simulink model "ESC"  (R2026b)
settings: Solver=FixedStepAuto  StopTime=1  FixedStep=1e-6
libraries: fl_lib x21, nesl_utility x18, ee_lib x8, simulink x2, slpidlib x1, eeGeneralControl x1
settings Model: Creator=aniru  LastModifiedBy=aniru
settings DebuggingCC: AlgebraicLoopMsg=none
settings SimscapeCC: SimscapeLogType=all  SimscapeNominalValues="[{\"value\":\"1\",\"unit\":\"A\"},{\"value\":\"1\",\"unit\":\"bar\"},{\"value\":\"1\",\"unit\":\"cm^2\"},{\"value\":\"1\",\"unit\":\"cm^3/s\"},{\"value\":\"1\",\"unit\":\"kJ/kg\"},{\"value\":\"1\",\"unit\":\"kW\"},{\"value\":\"1\",\"unit\":\"l\"},{\"value\":\"1\",\"unit\":\"N\"},{\"value\":\"1\",\"unit\":\"N*m\"},{\"value\":\"1\",\"unit\":\"V\"},{\"value\":\"0.001\",\"unit\":\"Wb\"}]"  SimscapeUseEnergyAccounting=off

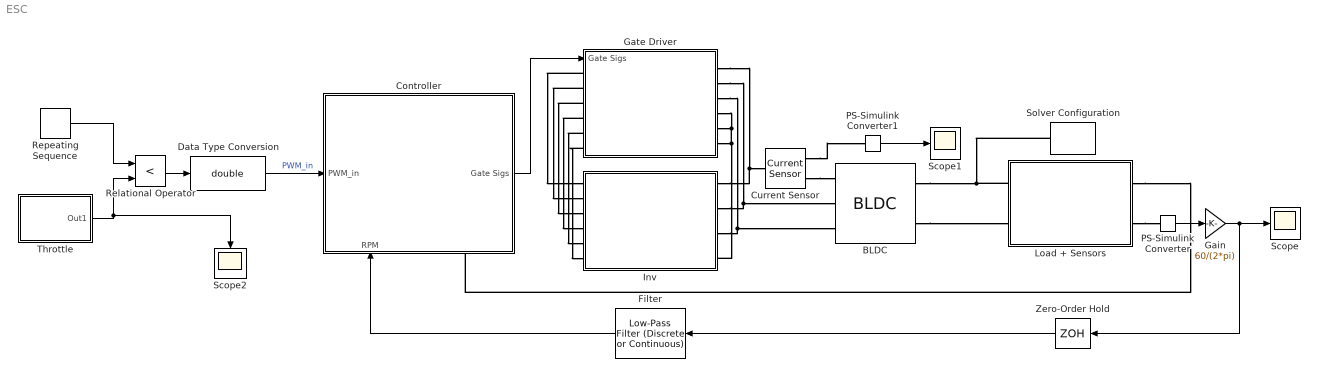
== system ESC ==
  BLDC : ee_lib/Electromechanical/Permanent Magnet/BLDC  PartSpecification="{\"CollectionId\":\"MW.SimscapeElectrical\",\"CollectionVersion\":\"1.0.0\",\"DatasetId\":\"Crouzet|80120301|simscape.electrical.bldc\",\"DisplayName\":\"Crouzet:80120301\"}"  rotor_param=ee.enum.pmsm.backemf.trapezoidflux  pm_flux_linkage=2.1333e-02 % Datasheet derived Wb  theta_constant=28.1250 % Assumed angle deg  emf_max=9.6 % Parameter not set V  w_meas=600 % Parameter not set rpm  DphiDtheta_tab=[0, -.1528, -.1528, .1528, .1528, 0] % Parameter not set Wb/rad  back_emf_tab=[0, -9.6, -9.6, 9.6, 9.6, 0] % Parameter not set V  rotor_angle_tab=[0, 7.5, 22.5, 37.5, 52.5, 60] % Parameter not set deg  nPolePairs=4 % Datasheet derived  axes_param=ee.enum.rotorangle.qaxis  port_option=ee.enum.threePhasePort.expanded  winding_type=ee.enum.electromech.statorconfiguration.wye  stator_param=ee.enum.statorparam.LdLqL0  machine_param=ee.enum.dqparameterization.constant  Ld=0.2300 % Datasheet derived mH  Lq=0.2300 % Datasheet derived mH  idVec=[-200, 0, 200] % Parameter not set A  iqVec=[-200, 0, 200] % Parameter not set A  LdMatrix=0.00022 * ones(3, 3) % Parameter not set H  LqMatrix=0.00022 * ones(3, 3) % Parameter not set H  L0=0.2300 % Assumed inductance value mH  Ls=0.0002 % Parameter not set H  Lm=0 % Parameter not set H  Ms=0.00002 % Parameter not set H  Rs=0.1000 % Datasheet derived Ohm  zero_sequence=ee.enum.park.zerosequence.exclude  loss_param=ee.enum.ironloss.none  losses_oc=[0, 0, 0] % Parameter not set W  losses_sc=[0, 0, 0] % Parameter not set W  f_losses=60 % Parameter not set Hz  Isc_losses=95 % Parameter not set A  J=1.6000e-04 % Datasheet derived kg*m^2  lam=0 % Parameter not set N*m*s/rad  i_d_specify=off  i_d_priority=None  i_d=0 A  i_d_nominal_specify=off  i_d_nominal_value=1  i_d_nominal_unit=A  i_q_specify=off  i_q_priority=None  i_q=0 A  i_q_nominal_specify=off  i_q_nominal_value=1  i_q_nominal_unit=A  torque_specify=off  torque_priority=None  torque=0 N*m  torque_nominal_specify=off  torque_nominal_value=1  torque_nominal_unit=N*m  angular_velocity_specify=off  angular_velocity_priority=High  angular_velocity=0 rpm  angular_velocity_nominal_specify=off  angular_velocity_nominal_value=1  angular_velocity_nominal_unit=rpm  angular_position_specify=off  angular_position_priority=High  angular_position=0 deg  angular_position_nominal_specify=off  angular_position_nominal_value=1  angular_position_nominal_unit=deg  alpha=3.93e-3 % Parameter not set 1/K  alpha_flux=-0.001 % Parameter not set 1/K  Tmeas=298.15 % Parameter not set K  stator_thermal_mass=100 % Parameter not set J/K  rotor_thermal_mass=200 % Parameter not set J/K  Rm_percent_rotor=90 % Parameter not set  Rd_percent_rotor=30 % Parameter not set  temperatureA_specify=off  temperatureA_priority=High  temperatureA=25 degC  temperatureA_nominal_specify=off  temperatureA_nominal_value=1  temperatureA_nominal_unit=degC  temperatureB_specify=off  temperatureB_priority=High  temperatureB=25 degC  temperatureB_nominal_specify=off  temperatureB_nominal_value=1  temperatureB_nominal_unit=degC  temperatureC_specify=off  temperatureC_priority=High  temperatureC=25 degC  temperatureC_nominal_specify=off  temperatureC_nominal_value=1  temperatureC_nominal_unit=degC  temperatureR_specify=off  temperatureR_priority=High  temperatureR=25 degC  temperatureR_nominal_specify=off  temperatureR_nominal_value=1  temperatureR_nominal_unit=degC
      settings: AttributesFormatString=Crouzet:80120301
  Controller : Subsystem
      settings: PortSchema="{\"entries\":[{\"content\":{\"sides\":[{\"content\":{\"connectorIds\":[\"In1\"]},\"type\":\"ConnectorPlacement.EquallySpacedRectSide\",\"uuid\":\"d20efde7-2380-411c-918f-9135c5284e68\"},{\"content\":{\"connectorIds\":[\"Out1\"],\"side\":\"RIGHT\"},\"type\":\"ConnectorPlacement.EquallySpacedRectSide\",\"uuid\":\"b87beafc-0c27-449f-9c72-bbb0e463092f\"},{\"content\":{\"side\":\"TOP\"},\"type\":\"ConnectorPlacement.EquallySpacedRectSide\",\"uuid\":\"b8d85be5-c3c9-47b7-b090-b5424d23e700\"},{\"content\":{\"connectorIds\":[\"In2\",\"RConn1\"],\"side\":\"BOTTOM\"},\"type\":\"ConnectorPlacement.EquallySpacedRectSide\",\"uuid\":\"c2a9ca41-a9b6-416c-a6db-c5c92e119f95\"}]},\"type\":\"ConnectorPlacement.EquallySpacedConnector\",\"uuid\":\"fe6135bb-2d05-4881-a2f1-961b4e6c139d\"}],\"packageUris\":[\"http://schema.mathworks.com/mf0/Connector/R2020b\"],\"version\":\"1.0\"}"
  Current Sensor : fl_lib/Electrical/Electrical Sensors/Current Sensor
  Data Type Conversion : DataTypeConversion  OutDataTypeStr=double  SaturateOnIntegerOverflow=off  RndMeth=Floor
  Filter : eeGeneralControl/Low-Pass Filter (Discrete or Continuous)  K=1  T=0.00318  B=inf  A=-inf  init_option=Inherited from block input  x0=0  Ts=-1
  Gain : Gain  Gain=60/(2*pi)
  Gate Driver : Subsystem
      settings: PortSchema="{\"entries\":[{\"content\":{\"sides\":[{\"content\":{\"connectorIds\":[\"LConn1\",\"LConn2\",\"LConn3\",\"LConn4\",\"LConn5\",\"LConn6\"]},\"type\":\"ConnectorPlacement.EquallySpacedRectSide\",\"uuid\":\"b49da606-eaf8-42ea-bde7-8db1abebf234\"},{\"content\":{\"connectorIds\":[\"In1\",\"RConn1\",\"RConn2\",\"RConn3\",\"RConn4\",\"RConn5\",\"RConn6\"],\"side\":\"RIGHT\"},\"type\":\"ConnectorPlacement.EquallySpacedRectSide\",\"uuid\":\"1a40fae2-693e-4820-81cb-e8ff43bbd20f\"},{\"content\":{\"side\":\"TOP\"},\"type\":\"ConnectorPlacement.EquallySpacedRectSide\",\"uuid\":\"e869c746-5bf4-4881-9f55-64e2cb76af97\"}]},\"type\":\"ConnectorPlacement.EquallySpacedConnector\",\"uuid\":\"eea107e6-2ce8-4a20-b51d-4fd136cf8702\"}],\"packageUris\":[\"http://schema.mathworks.com/mf0/Connector/R2020b\"],\"version\":\"1.0\"}"
  Inv : Subsystem
  Load + Sensors : Subsystem
  PS-Simulink Converter : nesl_utility/PS-Simulink Converter  PhysicalDomain=network_engine_domain  SubClassName=ps_output  LeftPortType=input  RightPortType=output  PseudoPeriodic=off  Frequencies=[]  VectorFormat=inherit  Unit=rad/s  AffineConversion=off
  PS-Simulink Converter1 : nesl_utility/PS-Simulink Converter  PhysicalDomain=network_engine_domain  SubClassName=ps_output  LeftPortType=input  RightPortType=output  PseudoPeriodic=off  Frequencies=[]  VectorFormat=inherit  Unit=inherit  AffineConversion=off
  Relational Operator : RelationalOperator  Operator=<  OutDataTypeStr=boolean  RndMeth=Simplest  InputSameDT=off
  Repeating Sequence : simulink/Sources/Repeating Sequence  rep_seq_t=[0 0.02]  rep_seq_y=[0 0.02]
  Scope : Scope
      settings: Title=SPEED vs Time  ActiveDisplayYMinimum=-450.81242260219108  ActiveDisplayYMaximum=1125.4093407717337  YLabel=RPM  DataLoggingMaxPoints=500000  DataLoggingDecimation=10  DataLoggingSaveFormat=Array
  Scope1 : Scope
      settings: ActiveDisplayYMinimum=-42.67051907682562  ActiveDisplayYMaximum=44.8132549409085  YLabel=Current (A phase)  DataLoggingMaxPoints=500000  DataLoggingDecimation=100  DataLoggingSaveFormat=Array
  Scope2 : Scope
      settings: ActiveDisplayYMinimum=0.00115  ActiveDisplayYMaximum=0.00165  YLabel=PWM_in  DataLoggingVariableName=ScopeData2  DataLoggingSaveFormat=Array
  Solver Configuration : nesl_utility/Solver Configuration  PhysicalDomain=network_engine_domain  SubClassName=solver  LeftPortType=input  RightPortType=generic  Tones=[]  Harmonics=[]  SimulateNoise=off  Profile=off  UseLocalSampling=off  EnableSwitchedLinearOptims=on  FrequencyDomain=off  UseCCode=off  RelTol=0.001  AbsTol=0.001  MinStep=1e-09  ToWorkspace=off  RevertToSquareIcSolve=off  NumHomotopyIterations=100  PhasorMode=off  PhasorModeNumHarmonics=1  ConsistencySolver=NEWTON_XTOL_AFTER_FTOL  CanonicalOrdering=CANONICAL  OptimizeIntermediates=OPTIMIZED  MulticoreSolverChoice=BACKWARD_EULER  IndexReductionMethod=DerivativeReplacement  DoDC=off  ResidualTolerance=1e-09  ConsistencyTolSource=GLOBAL  ConsistencyAbsTol=0.001  ConsistencyRelTol=0.001  ConsistencyTolFactor=0.001  UseLocalSolver=on  LocalSolverChoice=NE_BACKWARD_EULER_ADVANCER  ResolveIndetEquations=on  FunctionEvalNumThread=1  LocalSolverSampleTime=1e-6  DoFixedCost=on  MaxNonlinIter=3  MaxModeIter=2  ComputeImpulses=off  ImpulseIterations=2  LinearAlgebra=auto  LinearAlgebraNumThread=0  EquationFormulation=NE_TIME_EF  DelaysMemoryBudget=1024  AutomaticFiltering=on  FilteringTimeConstant=0.001  PartitionStorageMethod=AS_NEEDED  PartitionMemoryBudget=1024  PartitionMethod=BALANCED  MultibodyUseLocalSolver=off  MultibodyLocalSolverChoice=ODE1  MultibodyLocalSolverSampleTime=0.001
  Throttle : Subsystem
  Zero-Order Hold : ZeroOrderHold  SampleTime=1e-3
  wires:
  PS-Simulink Converter/1 -> Gain/1
  PS-Simulink Converter1/1 -> Scope1/1
  Gain/1 -> Scope/1, Zero-Order Hold/1
  Controller/1(Gate Sigs) -> Gate Driver/1(Gate Sigs)
  Repeating Sequence/1 -> Relational Operator/1
  Throttle/1(Out1) -> Scope2/1, Relational Operator/2
  Relational Operator/1 -> Data Type Conversion/1
  Data Type Conversion/1 -> Controller/1(PWM_in)  "PWM_in"
  Zero-Order Hold/1 -> Filter/1
  Filter/1 -> Controller/2(RPM)
  connections:
  Inv/RConn2 -- Gate Driver/LConn2 -- BLDC/LConn2
  Inv/RConn1 -- Gate Driver/LConn1 -- Current Sensor/LConn1
  Inv/RConn3 -- Gate Driver/LConn3 -- BLDC/LConn3
  Gate Driver/RConn1 -- Inv/LConn1
  Gate Driver/RConn2 -- Inv/LConn2
  Gate Driver/RConn3 -- Inv/LConn3
  Gate Driver/RConn4 -- Inv/LConn4
  Gate Driver/RConn5 -- Inv/LConn5
  Gate Driver/RConn6 -- Inv/LConn6
  Gate Driver/LConn6 -- Gate Driver/LConn4 -- Gate Driver/LConn5 -- Inv/RConn4
  BLDC/RConn1 -- Load + Sensors/LConn1 -- Solver Configuration/RConn1
  Current Sensor/RConn2 -- BLDC/LConn1
  Current Sensor/RConn1 -- PS-Simulink Converter1/LConn1
  BLDC/RConn2 -- Load + Sensors/LConn2
  Load + Sensors/RConn2 -- PS-Simulink Converter/LConn1
  Load + Sensors/RConn1 -- Controller/RConn1

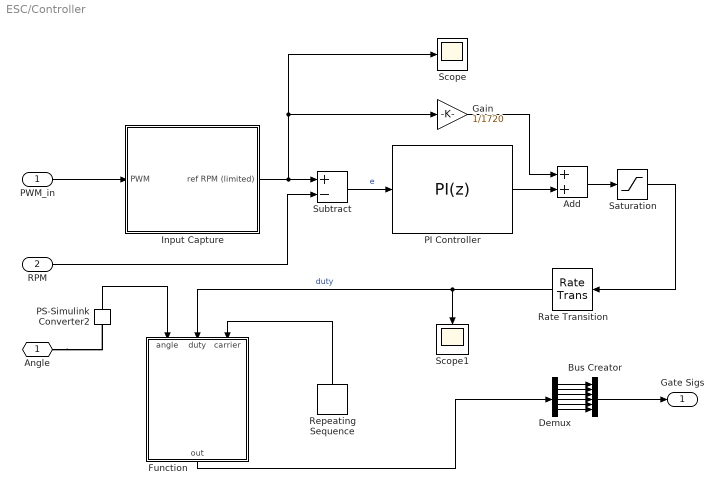
== system ESC/Controller ==
  PWM_in : Inport
  RPM : Inport  Port=2
  Add : Sum
  Bus Creator : BusCreator  Inputs=6
  Demux : Demux  Outputs=6
  Function : MATLAB Function  TreatAsAtomicUnit=on
  Gain : Gain  Gain=1/1720
  Input Capture : Subsystem
  PI Controller : slpidlib/PID Controller  Controller=PI  Form=Parallel  TimeDomain=Discrete-time  UseExternalTs=off  SampleTime=1e-3  IntegratorMethod=Forward Euler  FilterMethod=Forward Euler  ControllerParametersSource=internal  P=5e-4  I=2e-5  UseKiTs=on  D=0  UseExternalDerivativeSource=off  N=100  UseFilter=on  TunerSelectOption=Transfer Function Based (PID Tuner App)  ZeroCross=off  InitialConditionSource=internal  InitialConditionForIntegrator=0  InitialConditionForFilter=0  DifferentiatorICPrevScaledInput=0  ExternalReset=none  TrackingMode=off  Kt=1  LimitOutput=on  SatLimitsSource=internal  UpperSaturationLimit=0.5  LowerSaturationLimit=-0.5  LinearizeAsGain=on  AntiWindupMode=clamping  Kb=1  LimitIntegrator=off  UpperIntegratorSaturationLimit=0.5  LowerIntegratorSaturationLimit=-0.5  RndMeth=Simplest  POutMin=[]  POutMax=[]  IOutMin=[]  IOutMax=[]  DOutMin=[]  DOutMax=[]  NOutMin=[]  NOutMax=[]  SumOutMin=[]  SumOutMax=[]  SaturationOutDataTypeStr=Inherit: Inherit via back propagation  SaturationOutMin=[]  SaturationOutMax=[]  PParamMin=[]  PParamMax=[]  IParamMin=[]  IParamMax=[]  DParamMin=[]  DParamMax=[]  NParamMin=[]  NParamMax=[]  KbParamMin=[]  KbParamMax=[]  KtParamMin=[]  KtParamMax=[]  KbOutMin=[]  KbOutMax=[]  KtOutMin=[]  KtOutMax=[]  IntegratorOutMin=[]  IntegratorOutMax=[]  FilterOutMin=[]  FilterOutMax=[]  SumI1OutMin=[]  SumI1OutMax=[]  SumI2OutMin=[]  SumI2OutMax=[]  SumI3OutMin=[]  SumI3OutMax=[]  SumI4OutMin=[]  SumI4OutMax=[]  SumDOutMin=[]  SumDOutMax=[]  DifferentiatorOutMin=[]  DifferentiatorOutMax=[]  FilterDiffOutCoefMin=[]  FilterDiffOutCoefMax=[]  ReciprocalOutMin=[]  ReciprocalOutMax=[]  SumDenOutMin=[]  SumDenOutMax=[]  SumNumOutMin=[]  SumNumOutMax=[]  DivideOutMin=[]  DivideOutMax=[]  UdiffTsProdOutMin=[]  UdiffTsProdOutMax=[]  NTsProdOutMin=[]  NTsProdOutMax=[]  UintegralTsProdOutMin=[]  UintegralTsProdOutMax=[]  UngainTsProdOutMin=[]  UngainTsProdOutMax=[]  ClampingZeroOutDataTypeStr=Inherit: Inherit via back propagation  ClampingZeroOutMin=[]  ClampingZeroOutMax=[]  FilterDenConstantOutDataTypeStr=Inherit: Inherit via back propagation  FilterDenConstantOutMin=[]  FilterDenConstantOutMax=[]  PCopyOutDataTypeStr=Inherit: Inherit via back propagation  PCopyOutMin=[]  PCopyOutMax=[]  NCopyOutDataTypeStr=Inherit: Inherit via back propagation  NCopyOutMin=[]  NCopyOutMax=[]  IntegratorContinuousStateAttributes=''  IntegratorStateMustResolveToSignalObject=off  IntegratorRTWStateStorageClass=Auto  FilterContinuousStateAttributes=''  FilterStateMustResolveToSignalObject=off  FilterRTWStateStorageClass=Auto  ParallelPVariant=InternalParameters  IdealPVariant=Disabled  IVariant=InternalParameters  DVariant=Disabled  IntegratorVariant=Discrete  SatVariant=Enabled  AWVariant=DiscClampingParallel  PCopyVariant=Disabled  TRVariant=Disabled  FdbkBlocksVariant=Forward  IdealPFdbkVariant=Disabled  SatFdbkVariant=Disabled  DerivativeFilterVariant=Disabled  NVariant=Disabled  NCopyVariant=Disabled_SignalSpec  FilterICVariant=Disabled  IntegratorICVariant=InternalICs  ExternalResetVariant=Disabled  TRSumVariant=Passthrough  SumFdbkVariant=Disabled  SumVariant=Sum_PI  TsampFilterVariant=InternalTs  TsampNgainVariant=Passthrough  TsampIntegralVariant=Disabled_SignalSpec  ExternalSaturationOutDataTypeStr=Inherit: Same as second input  DerivativeSourceVariant=Disabled  PreIntVariant=InternalPreInt
      settings: LibrarySourceBlock=mcblib/Control/Induction Machine/Controllers/PI Controller
  PS-Simulink Converter2 : nesl_utility/PS-Simulink Converter  PhysicalDomain=network_engine_domain  SubClassName=ps_output  LeftPortType=input  RightPortType=output  PseudoPeriodic=off  Frequencies=[]  VectorFormat=inherit  Unit=rad  AffineConversion=off
  Rate Transition : RateTransition  OutPortSampleTimeOpt=Inherit
  Repeating Sequence : simulink/Sources/Repeating Sequence  rep_seq_t=[0 1e-4]  rep_seq_y=[0 1]
  Saturation : Saturate  UpperLimit=1  LowerLimit=0.15
  Scope : Scope
      settings: ActiveDisplayYMinimum=-118.14249999999997  ActiveDisplayYMaximum=1063.2825  YLabel=Ref RPM  DataLoggingMaxPoints=500000  DataLoggingDecimation=1000  DataLoggingVariableName=ScopeData3  DataLoggingSaveFormat=Array
  Scope1 : Scope
      settings: ActiveDisplayYMinimum=-0.0898767826107151  ActiveDisplayYMaximum=0.808891043496436  YLabel=Duty  DataLoggingMaxPoints=500000  DataLoggingDecimation=100  DataLoggingVariableName=ScopeData4  DataLoggingSaveFormat=Array
  Subtract : Sum  Inputs=+-
  Angle : PMIOPort  Side=Right
  Gate Sigs : Outport
  wires:
  Demux/1 -> Bus Creator/1
  PS-Simulink Converter2/1 -> Function/1(angle)
  Demux/4 -> Bus Creator/4
  Demux/5 -> Bus Creator/5
  Demux/3 -> Bus Creator/3
  Demux/6 -> Bus Creator/6
  Demux/2 -> Bus Creator/2
  Function/1(out) -> Demux/1
  Bus Creator/1 -> Gate Sigs/1
  PWM_in/1 -> Input Capture/1(PWM)
  Input Capture/1(ref RPM (limited)) -> Subtract/1, Scope/1, Gain/1
  RPM/1 -> Subtract/2
  Subtract/1 -> PI Controller/1  "e"
  Gain/1 -> Add/1
  PI Controller/1 -> Add/2
  Add/1 -> Saturation/1
  Saturation/1 -> Rate Transition/1
  Repeating Sequence/1 -> Function/3(carrier)
  Rate Transition/1 -> Function/2(duty), Scope1/1  "duty"
  connections:
  Angle/RConn1 -- PS-Simulink Converter2/LConn1

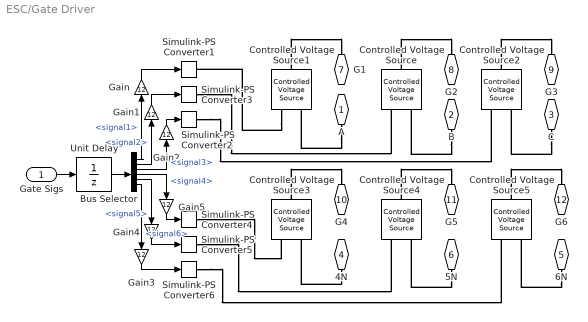
== system ESC/Gate Driver ==
  Gate Sigs : Inport
  Bus Selector : BusSelector  OutputSignals=signal1,signal2,signal3,signal4,signal5,signal6
  Controlled Voltage Source{,1..5} (6 alike) : fl_lib/Electrical/Electrical Sources/Controlled Voltage Source
  Gain{,1..5} (6 alike) : Gain  Gain=12
  Simulink-PS Converter{1..6} (6 alike) : nesl_utility/Simulink-PS Converter  PhysicalDomain=network_engine_domain  SubClassName=ps_input  LeftPortType=input  RightPortType=output  PseudoPeriodic=off  Frequencies=[]  NoiseDistribution=none  NoiseParameters=[]  Unit=1  AffineConversion=off  FilteringAndDerivatives=filter  SimscapeFilterOrder=1  InputFilterTimeConstant=1e-6  UdotUserProvided=0
  Unit Delay : UnitDelay  SampleTime=1e-6
  A : PMIOPort  Side=Left
  B : PMIOPort  Port=2  Side=Left
  C : PMIOPort  Port=3  Side=Left
  4N : PMIOPort  Port=4  Side=Left
  6N : PMIOPort  Port=5  Side=Left
  5N : PMIOPort  Port=6  Side=Left
  G1 : PMIOPort  Port=7  Side=Right
  G2 : PMIOPort  Port=8  Side=Right
  G3 : PMIOPort  Port=9  Side=Right
  G4 : PMIOPort  Port=10  Side=Right
  G5 : PMIOPort  Port=11  Side=Right
  G6 : PMIOPort  Port=12  Side=Right
  wires:
  Bus Selector/1 -> Gain/1  "<signal1>"
  Bus Selector/2 -> Gain1/1  "<signal2>"
  Bus Selector/5 -> Gain4/1  "<signal5>"
  Bus Selector/6 -> Gain3/1  "<signal6>"
  Gate Sigs/1 -> Unit Delay/1
  Gain/1 -> Simulink-PS Converter1/1
  Gain1/1 -> Simulink-PS Converter3/1
  Gain2/1 -> Simulink-PS Converter2/1
  Bus Selector/3 -> Gain2/1  "<signal3>"
  Gain3/1 -> Simulink-PS Converter6/1
  Gain4/1 -> Simulink-PS Converter5/1
  Gain5/1 -> Simulink-PS Converter4/1
  Bus Selector/4 -> Gain5/1  "<signal4>"
  Unit Delay/1 -> Bus Selector/1
  connections:
  Controlled Voltage Source/LConn1 -- G2/RConn1
  Simulink-PS Converter3/RConn1 -- Controlled Voltage Source/RConn1
  B/RConn1 -- Controlled Voltage Source/RConn2
  A/RConn1 -- Controlled Voltage Source1/RConn2
  Controlled Voltage Source1/RConn1 -- Simulink-PS Converter1/RConn1
  Controlled Voltage Source1/LConn1 -- G1/RConn1
  C/RConn1 -- Controlled Voltage Source2/RConn2
  Simulink-PS Converter2/RConn1 -- Controlled Voltage Source2/RConn1
  Controlled Voltage Source2/LConn1 -- G3/RConn1
  4N/RConn1 -- Controlled Voltage Source3/RConn2
  Simulink-PS Converter4/RConn1 -- Controlled Voltage Source3/RConn1
  Controlled Voltage Source3/LConn1 -- G4/RConn1
  5N/RConn1 -- Controlled Voltage Source4/RConn2
  Simulink-PS Converter5/RConn1 -- Controlled Voltage Source4/RConn1
  Controlled Voltage Source4/LConn1 -- G5/RConn1
  6N/RConn1 -- Controlled Voltage Source5/RConn2
  Simulink-PS Converter6/RConn1 -- Controlled Voltage Source5/RConn1
  Controlled Voltage Source5/LConn1 -- G6/RConn1

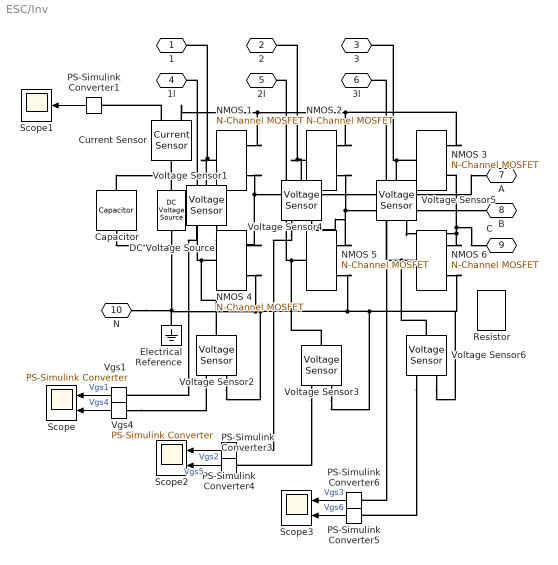
== system ESC/Inv ==
  Capacitor : fl_lib/Electrical/Electrical Elements/Capacitor  c=100 uF  r=1e-6 Ohm  g=0 1/Ohm  i_specify=off  i_priority=None  i=0 A  i_nominal_specify=off  i_nominal_value=1  i_nominal_unit=A  v_specify=off  v_priority=None  v=0 V  v_nominal_specify=off  v_nominal_value=1  v_nominal_unit=V  vc_specify=off  vc_priority=High  vc=0 V  vc_nominal_specify=off  vc_nominal_value=1  vc_nominal_unit=V
  Current Sensor : fl_lib/Electrical/Electrical Sensors/Current Sensor
  DC Voltage Source : fl_lib/Electrical/Electrical Sources/DC Voltage Source  v0=24 V
  Electrical Reference : fl_lib/Electrical/Electrical Elements/Electrical Reference
  NMOS {1..6} (6 alike) : ee_lib/Semiconductors & Converters/N-Channel MOSFET  paramTerminal=ee.enum.mosfet.numberOfTerminals.three  parameterization=ee.enum.mosfet.parameterization.datasheet  Beta=5.0 A/V^2  Rds=1 mOhm  Id=100 A  Vgs=10 V  Vth=3.5 V  Vth0=1.7 V  lam=0 1/V  gamma_vth=0.5 V^(1/2)  phib=0.5 V  Vth1=1.9071 V  Vbs1=-1 V  Vth2=2.066 V  Vbs2=-2 V  Tmeas=25 degC  Vgs_vec=[-1, -.5, 2, 3, 4, 5] V  Vds_vec=[0, 2, 4, 8, 12, 16, 20] V  Vbs_vec=[0, -4, -6, -12] V  T_vec=[25, 125] degC  Vth_vec=[.4, 1.2, 1.4, 1.45] V  Vth_mat=[.4, .35; 1.2, 1.15; 1.4, 1.35; 1.45, 1.4] V  Ids_mat=[0, 0, 0, 0, 0, 0, 0; 0, 0, 0, 0, 0, 0, 0; 0, .003, .0038, .0043, .0046, .0048, .0049; 0, .0055, .008, .009, .0095, .01, .0101; 0, .0115, .016, .018, .019, .0195, .02; 0, .0152, .0225, .0265, .028, .0295, .03] A  Ids_mat0=[0, 0, 0, 0, 0, 0, 0; 0, 0, 0, 0, 0, 0, 0; 0, .003, .0038, .0043, .0046, .0048, .0049; 0, .0055, .008, .009, .0095, .01, .0101; 0, .0115, .016, .018, .019, .0195, .02; 0, .0152, .0225, .0265, .028, .0295, .03] A  Ids_mat_3D=zeros(6, 7, 2) A  Ids_mat_3D0=zeros(6, 7, 2) A  IV_table_symmetry=ee.enum.mosfet.symmetricNIV.no  RS=0.0001 Ohm  RD=0 Ohm  RB=0.001 Ohm  LeadRs=0 Ohm  LeadRd=0 Ohm  LeadRg=2.1 Ohm  LeadRb=0 Ohm  LS=0 nH  LD=0 nH  LG=0 nH  LB=0 nH  C_param=ee.enum.mosfet.capacitanceParam.fixedciss  C_GS=270 pF  C_GD=80 pF  C_GB=0 pF  C_DS=0 pF  C_iss=14240 pF  C_rss=1460 pF  C_oss=2920 pF  C_iss_vec=[720, 700, 590, 470, 390, 310] pF  C_rss_vec=[450, 400, 300, 190, 95, 55] pF  C_oss_vec=[900, 810, 690, 420, 270, 170] pF  C_GS_vec=[270, 300, 290, 280, 295, 255] pF  C_GD_vec=[450, 400, 300, 190, 95, 55] pF  C_GB_vec=[270, 300, 290, 280, 295, 255] pF  C_Vgs_vec=0 V  C_DS_vec=[450, 410, 390, 230, 175, 115] pF  C_Vds_vec=[.1, .3, 1, 3, 10, 30] V  V_GS_for_cap_data=0 V  charge_linearity_param=ee.enum.mosfet.cgdLinearity.constant  C_OX=200 pF  V_C_OX=-0.5 V  charge_linearity_param_vgb=ee.enum.mosfet.cgbLinearity.instantly  charge_linearity_param_with_vgb=ee.enum.mosfet.cgbLinearityWithSeparateCgb.instantly  Di_param=ee.enum.mosfet.diodeParam.exponential  IsDiode=3.6e-13 A  Vbi=0.86 V  n=1  Cj0Diode=0 pF  TT=1e-9 s  Tmeas_dio=25 degC  TableTypeNoT=ee.enum.mosfet.tableType.IfMat  TableType=ee.enum.diode.tableType.IfMat  IfVec=[.07, .12, .19, 1.75, 4.24, 7.32, 11.2] A  IfMat=[.07, .12, .19, 1.75, 4.24, 7.32, 11.2; .16, .3, .72, 2.14, 4.02, 6.35, 9.12] A  VfVecV=[.9, 1.15, 1.25, 1.5, 1.75, 2.17, 2.6, 2.85] V  VfMatV=[.9, 1.15, 1.25, 1.5, 1.75, 2.17, 2.6, 2.85; .58, .68, .75, 1.1, 1.38, 1.77, 2.27, 2.7] V  TjVec=[25, 125] degC  VfVec=[.5, .7, .9, 1.3, 1.7, 2.1, 2.5] V  IfVecV=[.1, .2, .5, 1, 2, 4, 7, 10] A  diode_Goff=1e-12 1/Ohm  prmDatasheet=ee.enum.temperatureParameterization.none  prmEquCoeff=ee.enum.temperatureParameterization.none  dVth_dT=-6 mV/K  dVth0_dT=-6 mV/K  Rds_T2=0.037 Ohm  BEXDatasheet=-1.5  BEXEquCoeff=-1.5  etaisDatasheet=3  etaisEquCoeff=3  Tmeas2=125 degC  etaisTabulated=3  TdeviceDatasheet=25 degC  TdeviceEquCoeff=25 degC  TdeviceTabulated=25 degC  i_g_specify=off  i_g_priority=None  i_g=0 A  i_g_nominal_specify=off  i_g_nominal_value=1  i_g_nominal_unit=A  i_d_specify=off  i_d_priority=None  i_d=0 A  i_d_nominal_specify=off  i_d_nominal_value=1  i_d_nominal_unit=A  i_b_specify=off  i_b_priority=None  i_b=0 A  i_b_nominal_specify=off  i_b_nominal_value=1  i_b_nominal_unit=A  voltage_gs_specify=off  voltage_gs_priority=None  voltage_gs=0 V  voltage_gs_nominal_specify=off  voltage_gs_nominal_value=1  voltage_gs_nominal_unit=V  voltage_ds_specify=off  voltage_ds_priority=None  voltage_ds=0 V  voltage_ds_nominal_specify=off  voltage_ds_nominal_value=1  voltage_ds_nominal_unit=V  voltage_bs_specify=off  voltage_bs_priority=None  voltage_bs=0 V  voltage_bs_nominal_specify=off  voltage_bs_nominal_value=1  voltage_bs_nominal_unit=V  v_Cgs_specify=off  v_Cgs_priority=High  v_Cgs=0 V  v_Cgs_nominal_specify=off  v_Cgs_nominal_value=1  v_Cgs_nominal_unit=V  v_Cds_specify=off  v_Cds_priority=High  v_Cds=0 V  v_Cds_nominal_specify=off  v_Cds_nominal_value=1  v_Cds_nominal_unit=V  v_Cbs_specify=off  v_Cbs_priority=High  v_Cbs=0 V  v_Cbs_nominal_specify=off  v_Cbs_nominal_value=1  v_Cbs_nominal_unit=V  thermal_network_parameterization=ee.enum.thermalNetworkTopology.junctionCase  Rth=[0, 10] K/W  Rth_Cauer=[1, 3, 10] K/W  Rth_Foster=[.08, .14, .22, .16] K/W  thermal_mass_parameterization=ee.enum.thermalNetwork.timeconstant  thermal_mass=[0, 1] J/K  thermal_mass_Cauer=[.1, .3, 1] J/K  thermal_mass_Foster=[.001, .005, .05, .5] J/K  thermal_time_constant=[0, 10] s  thermal_time_constant_Cauer=[1, 3, 10] s  thermal_time_constant_Foster=[7e-05, .0007, .01, .08] s  thermal_mass_initial_temperatures=[25, 25] degC  thermal_mass_initial_temperatures_Cauer=[25, 25, 25] degC  Tvec_initial_Foster=[25, 25, 25, 25] degC  betaref=18 A/V^2  Vfbref=-1.1 V  gamma=3.5 V^(1/2)  phib2ref=1 V  thesatref=0.4 1/V  alpha=0  Vp=5e-2 V  thesrref=0 1/V  m=8  Tref=25 degC  Rsref=2e-3 Ohm  Rdref=0.17 Ohm  Rgref=8.4 Ohm  Rbref=2e-3 Ohm  Cox=1500 pF  Cgso=100 pF  Cgdo=14 pF  Isref=5.2e-13 A  Cj0=480 pF  Tprm=ee.enum.temperatureParameterization.none  etabet=1.3  Stvfb=5e-4 V/K  Stphib=-8.5e-4 V/K  etasat=1.04  etasr=0.65  etar=0.95  etais=3  Tsim=25 degC  Ig_specify=off  Ig_priority=None  Ig=0 A  Ig_nominal_specify=off  Ig_nominal_value=1  Ig_nominal_unit=nA  Ids_specify=off  Ids_priority=None  Ids=0 A  Ids_nominal_specify=off  Ids_nominal_value=1  Ids_nominal_unit=A  Ib_specify=off  Ib_priority=None  Ib=0 A  Ib_nominal_specify=off  Ib_nominal_value=1  Ib_nominal_unit=uA  V_gs_specify=off  V_gs_priority=None  V_gs=0 V  V_gs_nominal_specify=off  V_gs_nominal_value=1  V_gs_nominal_unit=V  V_ds_specify=off  V_ds_priority=None  V_ds=0 V  V_ds_nominal_specify=off  V_ds_nominal_value=1  V_ds_nominal_unit=V  V_bs_specify=off  V_bs_priority=None  V_bs=0 V  V_bs_nominal_specify=off  V_bs_nominal_value=1  V_bs_nominal_unit=V  QGoverCox_specify=off  QGoverCox_priority=None  QGoverCox=0 V  QGoverCox_nominal_specify=off  QGoverCox_nominal_value=1  QGoverCox_nominal_unit=V  QDoverCox_specify=off  QDoverCox_priority=None  QDoverCox=0 V  QDoverCox_nominal_specify=off  QDoverCox_nominal_value=1  QDoverCox_nominal_unit=V  QBoverCox_specify=off  QBoverCox_priority=None  QBoverCox=0 V  QBoverCox_nominal_specify=off  QBoverCox_nominal_value=1  QBoverCox_nominal_unit=V  T0=[25, 25] degC  T0_Cauer=[25, 25, 25] degC
  PS-Simulink Converter{1,3..6} (5 alike) : nesl_utility/PS-Simulink Converter  PhysicalDomain=network_engine_domain  SubClassName=ps_output  LeftPortType=input  RightPortType=output  PseudoPeriodic=off  Frequencies=[]  VectorFormat=inherit  Unit=inherit  AffineConversion=off
  Resistor : ee_lib/Passive/Resistor  R=1 kOhm  enable_R_tol=ee.enum.toleranceApplication.none  R_tol=5  tol_distribution=ee.enum.toleranceDistribution.uniform  nSigma=4  enable_operating_limits=ee.enum.enable.no  operating_limit_action=ee.enum.passive.reportOpLim.warn  power_rating=1 W  max_working_voltage=100 V  noise_mode=ee.enum.sources.noise.Disabled  Tdevice=25 degC  sample_time=1e-3 s  repeatability=ee.enum.ic.repeatability.notRepeatable  user_seed=0  auto_seed=3890346746  power_derating_T1=70 degC  power_derating_T2=155 degC  operating_temperature_range_vec=[-50, 150] degC  alpha=3.93e-3 1/K  Tmeas=25 degC  thermal_mass=100 J/K  temperature_specify=off  temperature_priority=High  temperature=298.15 K  temperature_nominal_specify=off  temperature_nominal_value=1  temperature_nominal_unit=K
  Scope : Scope  NumInputPorts=2
      settings: ActiveDisplayYMinimum=-1.4999999999999996  ActiveDisplayYMaximum=13.5  YLabel=Voltage  DataLoggingVariableName=ScopeData5
  Scope1 : Scope
      settings: ActiveDisplayYMinimum=-3630.9568139389162  ActiveDisplayYMaximum=6481.8983265342176  YLabel=Current  DataLoggingVariableName=ScopeData6
  Scope2 : Scope  NumInputPorts=2
      settings: ActiveDisplayYMinimum=-1.4999999999999996  ActiveDisplayYMaximum=13.5  YLabel=Voltage  DataLoggingVariableName=ScopeData8
  Scope3 : Scope  NumInputPorts=2
      settings: ActiveDisplayYMinimum=-1.4999999999999996  ActiveDisplayYMaximum=13.5  YLabel=Voltage  DataLoggingVariableName=ScopeData9
  Vgs1 : nesl_utility/PS-Simulink Converter  PhysicalDomain=network_engine_domain  SubClassName=ps_output  LeftPortType=input  RightPortType=output  PseudoPeriodic=off  Frequencies=[]  VectorFormat=inherit  Unit=inherit  AffineConversion=off
  Vgs4 : nesl_utility/PS-Simulink Converter  PhysicalDomain=network_engine_domain  SubClassName=ps_output  LeftPortType=input  RightPortType=output  PseudoPeriodic=off  Frequencies=[]  VectorFormat=inherit  Unit=inherit  AffineConversion=off
  Voltage Sensor{1..6} (6 alike) : fl_lib/Electrical/Electrical Sensors/Voltage Sensor
  1 : PMIOPort  Side=Left
  2 : PMIOPort  Port=2  Side=Left
  3 : PMIOPort  Port=3  Side=Left
  1l : PMIOPort  Port=4  Side=Left
  2l : PMIOPort  Port=5  Side=Left
  3l : PMIOPort  Port=6  Side=Left
  A : PMIOPort  Port=7  Side=Right
  B : PMIOPort  Port=8  Side=Right
  C : PMIOPort  Port=9  Side=Right
  N : PMIOPort  Port=10  Side=Right
  wires:
  Vgs4/1 -> Scope/2  "Vgs4"
  PS-Simulink Converter1/1 -> Scope1/1
  Vgs1/1 -> Scope/1  "Vgs1"
  PS-Simulink Converter4/1 -> Scope2/1  "Vgs2"
  PS-Simulink Converter3/1 -> Scope2/2  "Vgs5"
  PS-Simulink Converter5/1 -> Scope3/2  "Vgs6"
  PS-Simulink Converter6/1 -> Scope3/1  "Vgs3"
  connections:
  NMOS 2/RConn2 -- Voltage Sensor4/RConn2 -- NMOS 5/RConn1 -- B/RConn1
  Voltage Sensor6/RConn2 -- NMOS 6/RConn2 -- Voltage Sensor3/RConn2 -- NMOS 5/RConn2 -- Voltage Sensor2/RConn2 -- NMOS 4/RConn2 -- N/RConn1 -- Capacitor/RConn1 -- DC Voltage Source/RConn1 -- Electrical Reference/LConn1
  NMOS 1/RConn2 -- Voltage Sensor1/RConn2 -- NMOS 4/RConn1 -- A/RConn1
  NMOS 6/RConn1 -- Voltage Sensor5/RConn2 -- NMOS 3/RConn2 -- C/RConn1
  NMOS 1/LConn1 -- Voltage Sensor1/LConn1 -- 1/RConn1
  NMOS 2/LConn1 -- Voltage Sensor4/LConn1 -- 2/RConn1
  NMOS 3/LConn1 -- Voltage Sensor5/LConn1 -- 3/RConn1
  NMOS 4/LConn1 -- Voltage Sensor2/LConn1 -- 1l/RConn1
  NMOS 5/LConn1 -- Voltage Sensor3/LConn1 -- 2l/RConn1
  NMOS 6/LConn1 -- Voltage Sensor6/LConn1 -- 3l/RConn1
  NMOS 1/RConn1 -- Current Sensor/RConn2 -- NMOS 3/RConn1 -- NMOS 2/RConn1
  Current Sensor/LConn1 -- Capacitor/LConn1 -- DC Voltage Source/LConn1
  Current Sensor/RConn1 -- PS-Simulink Converter1/LConn1
  Voltage Sensor1/RConn1 -- Vgs1/LConn1
  Vgs4/LConn1 -- Voltage Sensor2/RConn1
  Voltage Sensor4/RConn1 -- PS-Simulink Converter4/LConn1
  Voltage Sensor3/RConn1 -- PS-Simulink Converter3/LConn1
  Voltage Sensor5/RConn1 -- PS-Simulink Converter6/LConn1
  Voltage Sensor6/RConn1 -- PS-Simulink Converter5/LConn1

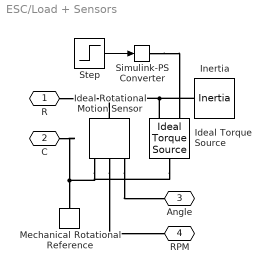
== system ESC/Load + Sensors ==
  Ideal Rotational Motion Sensor : fl_lib/Mechanical/Mechanical Sensors/Ideal Rotational Motion Sensor  reference=foundation.enum.MeasurementReference.difference  acceleration_port=false  velocity_port=true  position_port=true  wrap_angle=false  offset=0 rad
  Ideal Torque Source : fl_lib/Mechanical/Mechanical Sources/Ideal Torque Source
  Inertia : fl_lib/Mechanical/Rotational Elements/Inertia  inertia=1e-3 kg*m^2  num_ports=foundation.enum.numPorts2.one  w_specify=off  w_priority=High  w=0 rad/s  w_nominal_specify=off  w_nominal_value=1  w_nominal_unit=rad/s  t_specify=off  t_priority=None  t=0 N*m  t_nominal_specify=off  t_nominal_value=1  t_nominal_unit=N*m
  Mechanical Rotational Reference : fl_lib/Mechanical/Rotational Elements/Mechanical Rotational Reference
  Simulink-PS Converter : nesl_utility/Simulink-PS Converter  PhysicalDomain=network_engine_domain  SubClassName=ps_input  LeftPortType=input  RightPortType=output  PseudoPeriodic=off  Frequencies=[]  NoiseDistribution=none  NoiseParameters=[]  Unit=N*m  AffineConversion=off  FilteringAndDerivatives=provide  SimscapeFilterOrder=1  InputFilterTimeConstant=0.001  UdotUserProvided=0
  Step : Step  Time=0.2  InitialValue=0.5  FinalValue=1.5  SampleTime=0
  R : PMIOPort  Side=Left
  C : PMIOPort  Port=2  Side=Left
  Angle : PMIOPort  Port=3  Side=Right
  RPM : PMIOPort  Port=4  Side=Right
  wires:
  Step/1 -> Simulink-PS Converter/1
  connections:
  Inertia/LConn1 -- Ideal Torque Source/RConn2 -- R/RConn1 -- Ideal Rotational Motion Sensor/LConn1
  Ideal Rotational Motion Sensor/RConn2 -- RPM/RConn1
  Ideal Rotational Motion Sensor/RConn3 -- Angle/RConn1
  C/RConn1 -- Ideal Torque Source/LConn1 -- Ideal Rotational Motion Sensor/RConn1 -- Mechanical Rotational Reference/LConn1
  Simulink-PS Converter/RConn1 -- Ideal Torque Source/RConn1

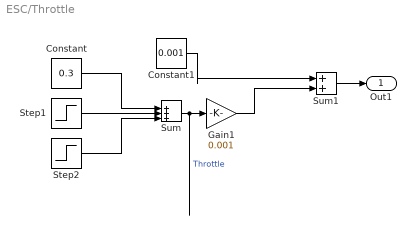
== system ESC/Throttle ==
  Constant : Constant  Value=0.3
  Constant1 : Constant  Value=0.001
  Gain1 : Gain  Gain=0.001
  Step1 : Step  Time=0.3  FinalValue=0.3  SampleTime=0
  Step2 : Step  Time=0.6  FinalValue=-0.4  SampleTime=0
  Sum : Sum  Inputs=|+++
  Sum1 : Sum  Inputs=|++
  Out1 : Outport
  wires:
  Constant1/1 -> Sum1/1
  Sum1/1 -> Out1/1
  Step2/1 -> Sum/3
  Constant/1 -> Sum/1
  Sum/1 -> Gain1/1  "Throttle"
  Step1/1 -> Sum/2
  Gain1/1 -> Sum1/2

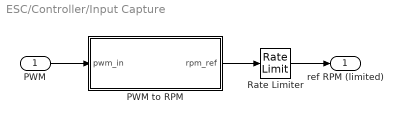
== system ESC/Controller/Input Capture ==
  PWM : Inport
  PWM to RPM : MATLAB Function  TreatAsAtomicUnit=on
  Rate Limiter : RateLimiter  RisingSlewLimit=3000  FallingSlewLimit=-6000  SampleTimeMode=inherited  InitialCondition=260
  ref RPM (limited) : Outport
  wires:
  PWM/1 -> PWM to RPM/1(pwm_in)
  PWM to RPM/1(rpm_ref) -> Rate Limiter/1
  Rate Limiter/1 -> ref RPM (limited)/1

== matlab function ESC/Controller/Input Capture/PWM to RPM ==
  settings: updateMethod=DISCRETE
  data: pwm_in input; rpm_ref output
function rpm_ref = fcn(pwm_in)
Ts = 1e-6;  RPM_MAX = 1400;           % rated speed
RPM_MIN = 260;                         % lowest commanded speed (duty ~0.15)

persistent cnt prev ref
if isempty(cnt), cnt = 0; prev = 0; ref = 0; end

if pwm_in > 0.5
    cnt = cnt + 1;
elseif prev > 0.5                      % falling edge: latch the width
    w = cnt*Ts;
    thr = min(max((w - 1e-3)/1e-3, 0), 1);
    if thr < 0.03
        ref = 0;                                   % stop
    else
        ref = RPM_MIN + thr*(RPM_MAX - RPM_MIN);   % map 0..1 to 260..1400
    end
    cnt = 0;
end
prev = pwm_in;
rpm_ref = ref;
end

== matlab function ESC/Controller/Function ==
  settings: updateMethod=DISCRETE  sampleTime=1e-6
  data: angle input; out output; duty input; carrier input
function out = fcn(angle, duty, carrier)
% Six-step commutation with complementary PWM, duty limits and full-on mode
% out = [G1 G2 G3 G4 G5 G6]'  (G1-3 = A,B,C high side; G4-6 = A,B,C low side)

Np     = 4;              % pole pairs (datasheet)
offset = 2*pi/6;         % your tuned electrical offset

% PWM limits (carrier must be 10 kHz: period 1e-4)
T_pwm     = 1e-4;
t_min_off = 15e-6;       % minimum complementary window
t_min_on  = 5e-6;        % minimum on-pulse
duty_max  = 1 - t_min_off/T_pwm;   % 0.85
duty_min  = t_min_on/T_pwm;        % 0.05

persistent pwm_prev
if isempty(pwm_prev), pwm_prev = 0; end

% Sector from rotor angle
theta_e = mod(Np*angle + offset, 2*pi);
s = floor(theta_e/(pi/3)) + 1;
s = min(max(s,1),6);

% Commutation table: columns G1 G2 G3 G4 G5 G6
T = [1 0 0 0 1 0;    % sector 1: A+ B-
    1 0 0 0 0 1;    % sector 2: A+ C-
    0 1 0 0 0 1;    % sector 3: B+ C-
    0 1 0 1 0 0;    % sector 4: B+ A-
    0 0 1 1 0 0;    % sector 5: C+ A-
    0 0 1 0 1 0];   % sector 6: C+ B-
g = T(s,:)';

% PWM with duty limits
if duty > duty_max
    pwm = 1;                         % full-on: no chopping
elseif duty < duty_min
    pwm = 0;                         % below minimum pulse: no on-time
else
    pwm = double(duty > carrier);
end

% One-sample dead time (1 us at Ts = 1e-6)
main = pwm * pwm_prev;               % chopped low switch
comp = (1 - pwm) * (1 - pwm_prev);   % complementary high switch
pwm_prev = pwm;

% Apply to the leg whose low side is active in this sector
for k = 1:3
    if g(3+k) == 1
        g(3+k) = main;   % low side chops
        g(k)   = comp;   % high side of the same leg, complementary
    end
end

out = g;
end
